simulink model "case_18_check_stopped"  (R2025b)
settings: Solver=VariableStepAuto  StartTime=0.0  StopTime=180  RelTol=1e-3
settings Model: Creator=sanborkl  LastModifiedBy=sanborkl

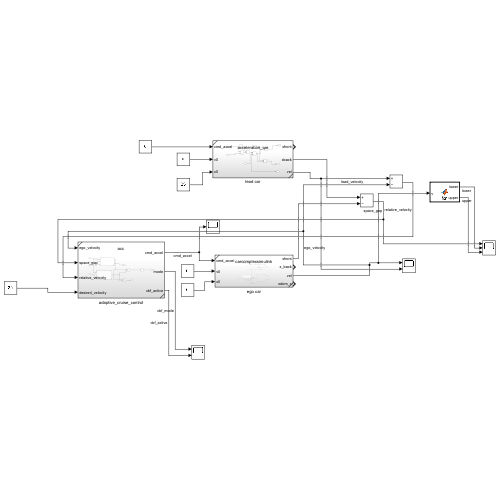
[thumbnail: Simulink's stored preview of the top-level diagram]
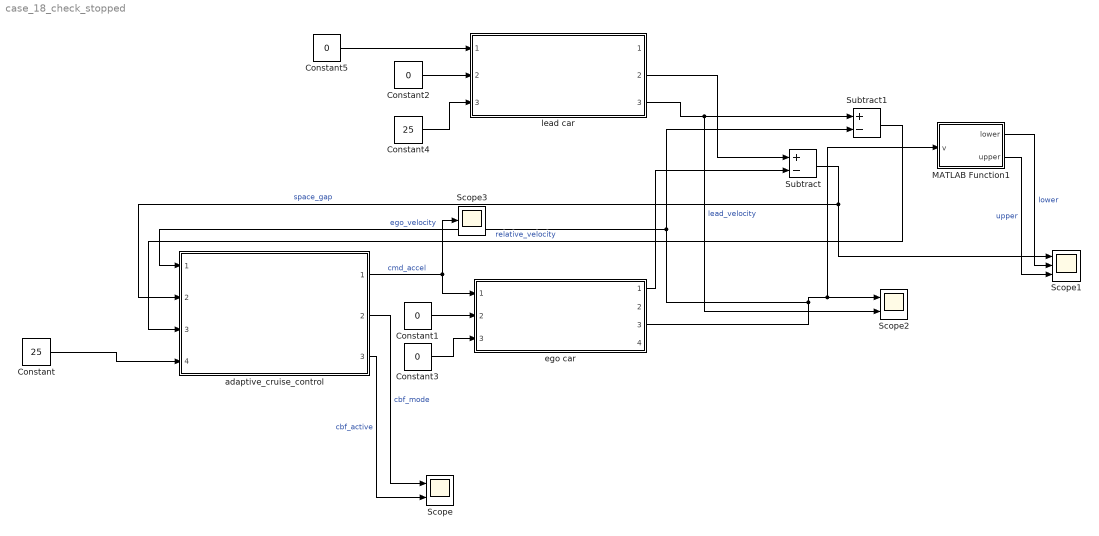
== system case_18_check_stopped ==
  Constant : Constant  Value=25
  Constant{1..3,5} (4 alike) : Constant  Value=0
  Constant4 : Constant  Value=25
  MATLAB Function1 : MATLAB Function  TreatAsAtomicUnit=on
  Scope : Scope  NumInputPorts=2
      settings: ActiveDisplayYMinimum=0.875  ActiveDisplayYMaximum=2.125
  Scope1 : Scope  NumInputPorts=3
      settings: ActiveDisplayYMinimum=3.0299626502234047  ActiveDisplayYMaximum=22.730004149975173  YLabel=m
  Scope2 : Scope  NumInputPorts=2
      settings: ActiveDisplayYMinimum=-0.13373381580762647  ActiveDisplayYMaximum=1.2036043422686384  YLabel=m/s  DataLoggingVariableName=ScopeData2
  Scope3 : Scope
      settings: ActiveDisplayYMinimum=-1.1898370540027552  ActiveDisplayYMaximum=0.70851688612408725  YLabel=m/s^2  DataLoggingVariableName=ScopeData3
  Subtract : Sum  Inputs=+-
  Subtract1 : Sum  Inputs=+-
  adaptive_cruise_control : Subsystem  ReferencedSubsystem=acc
  ego car : Subsystem  ReferencedSubsystem=carcomplexsimulink
  lead car : Subsystem  ReferencedSubsystem=acceleration_car
  wires:
  ego car/3 -> Scope2/1, MATLAB Function1/1(v), Subtract1/2, adaptive_cruise_control/1  "ego_velocity"
  adaptive_cruise_control/1 -> ego car/1, Scope3/1  "cmd_accel"
  Constant1/1 -> ego car/2
  Subtract1/1 -> adaptive_cruise_control/3  "relative_velocity"
  lead car/3 -> Scope2/2, Subtract1/1  "lead_velocity"
  Constant3/1 -> ego car/3
  Constant2/1 -> lead car/2
  adaptive_cruise_control/2 -> Scope/1  "cbf_mode"
  lead car/2 -> Subtract/1
  adaptive_cruise_control/3 -> Scope/2  "cbf_active"
  Constant/1 -> adaptive_cruise_control/4
  ego car/1 -> Subtract/2
  Subtract/1 -> Scope1/1, adaptive_cruise_control/2  "space_gap"
  Constant4/1 -> lead car/3
  Constant5/1 -> lead car/1
  MATLAB Function1/1(lower) -> Scope1/2  "lower"
  MATLAB Function1/2(upper) -> Scope1/3  "upper"

== matlab function case_18_check_stopped/MATLAB Function1 ==
  data: v input; lower output; upper output
function [lower, upper] = fcn(v)

lower = 2 * v + 5;
upper = 2 * v + 15;
